simulink model "model_Lab1"  (R2023b)
settings: Solver=VariableStepAuto  StartTime=0.0  StopTime=10.0  RelTol=1e-3
model workspace (MAT data in the model file):
  K1 = -1.9731
  Kp = -20
  tau = 0.02387
settings Model: Creator=micha  LastModifiedBy=micha

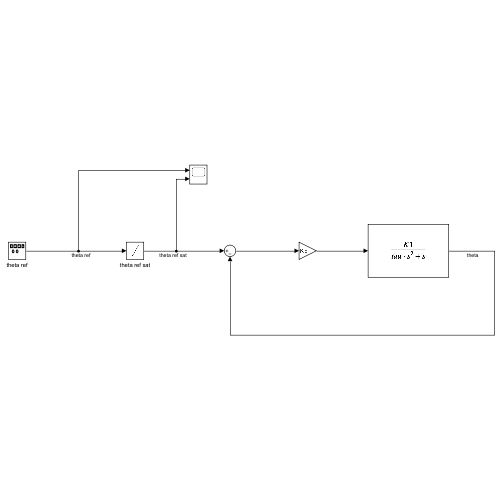
[thumbnail: Simulink's stored preview of the top-level diagram]
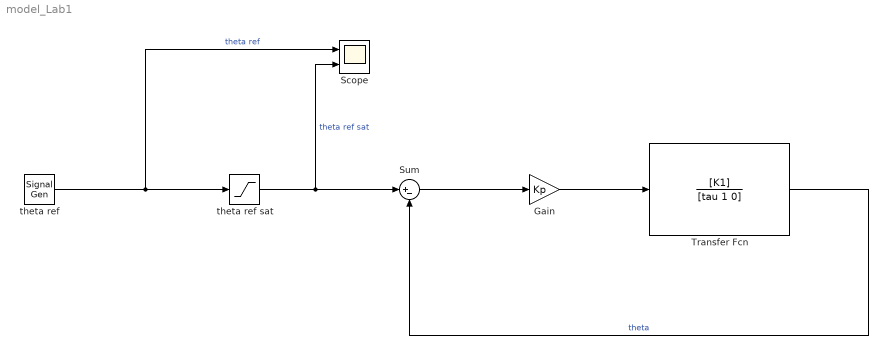
== system model_Lab1 ==
  Gain : Gain  Gain=Kp
  Scope : Scope  NumInputPorts=2
  Sum : Sum  Inputs=|+-
  Transfer Fcn : TransferFcn  Numerator=[K1]  Denominator=[tau 1 0]
  theta ref : SignalGenerator  WaveForm=square
  theta ref sat : Saturate  UpperLimit=0.7  LowerLimit=-0.7
  wires:
  theta ref/1 -> theta ref sat/1, Scope/1  "theta ref"
  theta ref sat/1 -> Sum/1, Scope/2  "theta ref sat"
  Sum/1 -> Gain/1
  Gain/1 -> Transfer Fcn/1
  Transfer Fcn/1 -> Sum/2  "theta"
